simulink model "Model_B"  (R2024b)
settings: Solver=ode15s  StartTime=0.0  StopTime=3  MaxStep=0.00020000000000000001  MinStep=1e-9  RelTol=9.9999999999999995e-08  AbsTol=1.0000000000000001e-09
PostLoadFcn:
  | f=fileparts(get_param(bdroot,'FileName'));addpath(f,fullfile(f,'..','ModelA'));
InitFcn:
  | Model_B_initialize(bdroot);
model workspace (MAT data in the model file):
  ic.Vnom = 1
  ic.referenceA.x0 = [0.0487207667186; 0; 1.03532101344; 2.70319926687e-24]
  ic.referenceA.V0 = 0.998847335682-0.048i
  ic.referenceA.Vnom = 1
  ic.referenceA.network = [0.998847335682; -0.048; 1; 1; 0.414093240727; 1.04542083745; 0.30480276799; 39666.4759309; 0; 1.22124532709e-15; 12.929734979; 0]
  ic.referenceA.residual = 1.21569421196e-14
  ic.referenceA.eigenvalues = [-0.599279843882+14.9008401777i; -0.599279843882-14.9008401777i; -5.25574712927+0i; -62.8318530718+0i]
  ic.x0 = [0.200769576757; 0; 1.03524949847; 1.07980110806e-24; 0; 0; 5.29655064166e-05; -1.84134158413e-05; 0.965950721518; -0.335811993898; 1.03524949847; -1.04303465943e-24; 0.965950721518; -0.404138460797]
  ic.y0 = [0.95847228581; -0.0493156664303; 0.959740151093; 0.95847228581; -0.0493156664303; 0.959740151093; 0.969798975745; -0.142871915924; 205.357045203; 0; 5.55111512313e-17; 2.71009793582; 0.994518056541; 0.144286965879; 1.04708580923; 1.03524949847; -1.04303465943e-24; 0.965950721518; -0.335811993898; 1.09045105116; 0.143213548258; 0; 0; 0; 0; 0]
  ic.residual = 1.79625227647e-12
  ic.Jacobian = [0  376.991118431  0  0  0  0  0  0  0  0  0  0  0  0; 0  -1.19464797706  -0.19232851257  0  0  0  0  0  0  0  0  0  -0.206126453186  0; 0  0  -5.03367820511  0  0  0  0  0  0  0  0  0  0  0.0862707915375; 0  0  0  -62.8318530718  0  0  0  0  0  0  0  0  0  0; 0  0  1.00000000001  -0.404138460697  0  0  0  0  0  0  -1.00000000001  0  0  0; 0  0  0  -0.965950721518  0  0  0  0  0  0  0  -1  -1.07980110809e-24  0; 0  0  0.00483446526552  -0.00195379334933  0.00172522007791  0  0  0  -1.00000000002  0  -0.00483446526552  -0.0660000000208  1.00000000002  0; 0  0.068326466901  0  -0.00466985516923  0  0.00172522013342  0  0  0  -1.00000000001  0.0660000000111  -0.00483446527255  0  0.999999999989; 0  -4.35983562251e-08  80.8855152144  -32.6889475634  28.8646844728  0  229177.356794  0  -16743.582286  7.83314234475e-08  -80.8855152144  -1104.24705101  16731.0159154  0; 0  1143.17120514  0  -78.1314211307  0  28.8646855192  0  229177.356794  0  -16743.5822859  1104.24705059  -80.8855154117  0  16731.0159149; 0  -3.93214802855e-22  0  0  0  0  0  0  5711.98664298  0  0  376.991118431  -5711.98664298  0; 0  -390.279866255  0  0  0  0  0  0  0  5711.98664293  -376.991118436  0  0  -5711.98664283; 1330.57569228  -152.356610329  0  0  0  0  0  0  0  0  2513.27412289  0  -171.394474141  1449.18654791; 2276.91091453  -364.154842827  0  0  0  0  0  0  0  0  0  2513.27412287  -1153.65532456  146.261732879]
  ic.eigenvalues = [-15794.2331673+321.061333144i; -15794.2331673-321.061333144i; -929.230478464+1324.15474358i; -929.230478464-1324.15474358i; -1.19066242403+12.8639119334i; -1.19066242403-12.8639119334i; -18.1217144526+11.723297357i; -18.1217144526-11.723297357i; -5.2077916342+0i; -13.5205584626+0.471109259308i; -13.5205584626-0.471109259308i; -0.361420035876+0i; -0.363265507273+0i; -62.8318530718+0i]
  networkParameters = [0.1; 0; 0.24; 1.2; 0.3; 1; 0; 0.01; 0; 1; 1]
  p.baseMVA = 100
  p.freq = 60
  p.M = 5.0224
  p.D = 6
  p.K = 12
  p.Dq = 60
  p.xe = 0.1
  p.xL1 = 0
  p.xL2 = 0.24
  p.PL = 1.2
  p.QL = 0.3
  p.VS = 1
  p.thetaS = 0
  p.Pref = 1
  p.Eref = 1.03532101344
  p.Qref = 0.414093240727
  p.Ithresh = 1.1
  p.Imax = 1.5
  p.SigmaXR = 5
  p.Vmax = 1
  p.KVI = 0.283333333333
  p.omegaVI = 62.8318530718
  p.xvmax = 0.566666666667
  p.faultEnabled = 1
  p.tFault = 0.1
  p.tClear = 0.18
  p.Rf = 0.01
  p.Xf = 0
  p.faultLoadToZ = 1
  p.Vswitch = 1
  p.tStop = 3
  p.solver = 'ode15s'
  p.maxStep = 0.0002
  p.relTol = 1e-07
  p.absTol = 1e-09
  p.initTol = 1e-09
  p.residualTol = 1e-07
  p.showFigures = 1
  p.saveResults = 1
  p.outputDir = 'D:\matlab\威\威-1304-售后-200-10.20\PI优化_20261020\ModelA\Model_A_results'
  p.basekV = 345
  p.xLf = 0.15
  p.xLc = 0.15
  p.bCf = 0.066
  p.rLf = 0.005
  p.rLc = 0.005
  p.Kpv = 0.00483446524834
  p.Kiv = 0.00172522012549
  p.Kpc = 6.65705971459
  p.Kic = 91.1867729461
  p.designCurrentHz = 3000
  p.designVoltageHz = 0.5
  p.designDamping = 4
values from neighbouring files (symbols this model uses):
  ic = Model_B_initial_state(p);mw.assignin('p',p);mw.assignin('ic',ic)    [Model_B_initialize.m]
  p = mw.getVariable('p')    [Model_B_initialize.m]    (also in Model_B_parameters.m = design_Model_B_PI(p,3000,.5,4); optimize_Model_B_PI.m = p0;for j=1:4,p.(names{j})=gains(j);end; refine_PI_local.m = p0;for gainIndex=1:4,p.(names{gainIndex})=gains(gainIndex);e)
settings Model: Creator=Administrator  LastModifiedBy=Administrator
settings DataIOCC: SaveOutput=off  SignalLogging=off
settings DebuggingCC: AlgebraicLoopMsg=error  MinStepSizeMsg=error

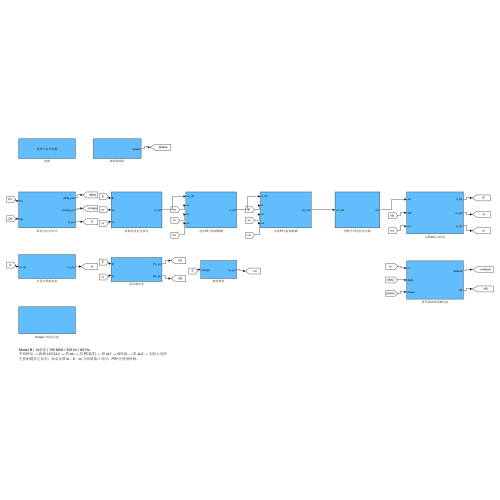
[thumbnail: Simulink's stored preview of the top-level diagram]
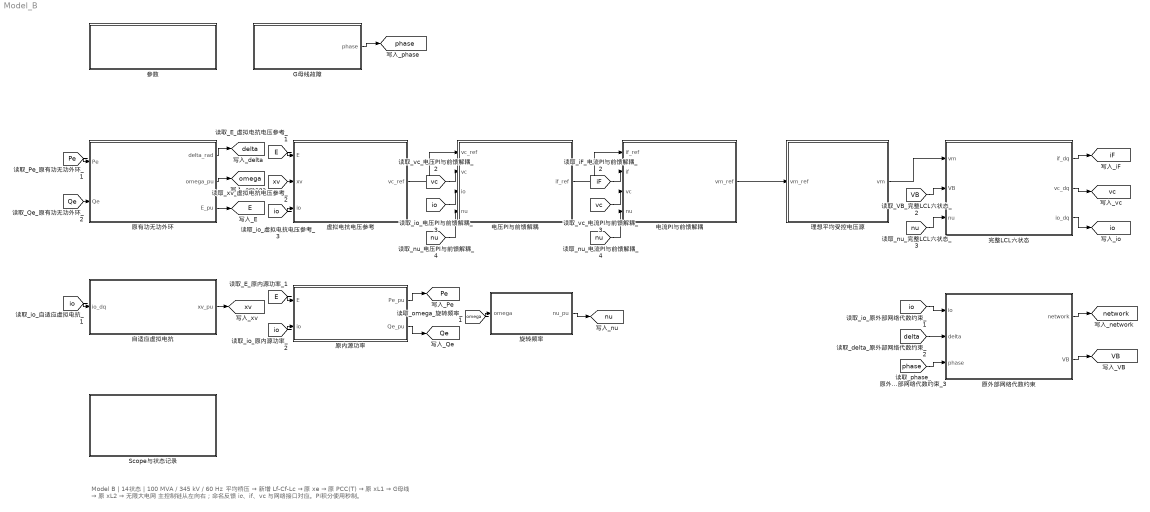
== system Model_B ==
  note: Model B | 14状态 | 100 MVA / 345 kV / 60 Hz
      | 平均桥压 → 新增 Lf-Cf-Lc → 原 xe → 原 PCC(T) → 原 xL1 → G母线 → 原 xL2 → 无限大电网
      | 主控制链从左向右；命名反馈 io、if、vc 与网络接口对应。PI积分使用秒制。
  G母线故障 : Subsystem
  Scope与状态记录 : Subsystem
  原内源功率 : Subsystem
  原外部网络代数约束 : Subsystem
  原有功无功外环 : Subsystem
  参数 : Subsystem  mask{baseMVA=100, freq=60, M=5.0224000000000002, D=6, K=12, Dq=60, xe=0.10000000000000001, xL1=0, xL2=0.23999999999999999, PL=1.2, QL=0.29999999999999999, VS=1, thetaS=0, Pref=1, Eref=1.0353210134405997, Qref=0.41409324072705855, Ithresh=1.1000000000000001, Imax=1.5, SigmaXR=5, Vmax=1, KVI=0.28333333333333344, omegaVI=62.831853071795862, xvmax=0.56666666666666676, faultEnabled=1, tFault=0.10000000000000001, tClear=0.17999999999999999, Rf=0.01, Xf=0, faultLoadToZ=1, Vswitch=1, tStop=3, maxStep=0.00020000000000000001, relTol=9.9999999999999995e-08, absTol=1.0000000000000001e-09, initTol=1.0000000000000001e-09, residualTol=9.9999999999999995e-08, basekV=345, xLf=0.14999999999999999, xLc=0.14999999999999999, bCf=0.066000000000000003, rLf=0.0050000000000000001, rLc=0.0050000000000000001, Kpv=0.0048344652483415206, Kiv=0.0017252201254877612, Kpc=6.6570597145874624, Kic=91.186772946123014}
      mask help: 标幺量与秒制。修改参数后直接运行，初值自动重新求解。
      mask Display: disp('系统与内环参数')
  完整LCL六状态 : Subsystem
  旋转频率 : Subsystem
  理想平均受控电压源 : Subsystem
  电压PI与前馈解耦 : Subsystem
  电流PI与前馈解耦 : Subsystem
  自适应虚拟电抗 : Subsystem
  虚拟电抗电压参考 : Subsystem
  tag scope: E=global, Pe=global, Qe=global, VB=global, delta=global, iF=global, io=global, network=global, nu=global, omega=global, phase=global, vc=global, xv=global
  wires:
  G母线故障/1(phase) -> [phase]
  [Pe] -> 原有功无功外环/1(Pe)
  [Qe] -> 原有功无功外环/2(Qe)
  原有功无功外环/1(delta_rad) -> [delta]
  原有功无功外环/2(omega_pu) -> [omega]
  原有功无功外环/3(E_pu) -> [E]
  [io] -> 自适应虚拟电抗/1(io_dq)
  自适应虚拟电抗/1(xv_pu) -> [xv]
  [E] -> 虚拟电抗电压参考/1(E)
  [xv] -> 虚拟电抗电压参考/2(xv)
  [io] -> 虚拟电抗电压参考/3(io)
  虚拟电抗电压参考/1(vc_ref) -> 电压PI与前馈解耦/1(vc_ref)
  [vc] -> 电压PI与前馈解耦/2(vc)
  [io] -> 电压PI与前馈解耦/3(io)
  [nu] -> 电压PI与前馈解耦/4(nu)
  电压PI与前馈解耦/1(if_ref) -> 电流PI与前馈解耦/1(if_ref)
  [iF] -> 电流PI与前馈解耦/2(if)
  [vc] -> 电流PI与前馈解耦/3(vc)
  [nu] -> 电流PI与前馈解耦/4(nu)
  电流PI与前馈解耦/1(vm_ref) -> 理想平均受控电压源/1(vm_ref)
  理想平均受控电压源/1(vm) -> 完整LCL六状态/1(vm)
  [VB] -> 完整LCL六状态/2(VB)
  [nu] -> 完整LCL六状态/3(nu)
  完整LCL六状态/1(if_dq) -> [iF]
  完整LCL六状态/2(vc_dq) -> [vc]
  完整LCL六状态/3(io_dq) -> [io]
  [io] -> 原外部网络代数约束/1(io)
  [delta] -> 原外部网络代数约束/2(delta)
  [phase] -> 原外部网络代数约束/3(phase)
  原外部网络代数约束/1(network) -> [network]
  原外部网络代数约束/2(VB) -> [VB]
  [E] -> 原内源功率/1(E)
  [io] -> 原内源功率/2(io)
  原内源功率/1(Pe_pu) -> [Pe]
  原内源功率/2(Qe_pu) -> [Qe]
  [omega] -> 旋转频率/1(omega)
  旋转频率/1(nu_pu) -> [nu]

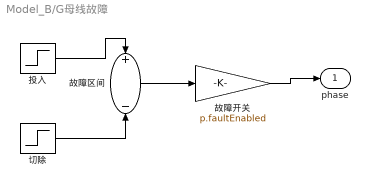
== system Model_B/G母线故障 ==
  切除 : Step  Time=p.tClear  SampleTime=0
  投入 : Step  Time=p.tFault  SampleTime=0
  故障区间 : Sum  Inputs=+-
  故障开关 : Gain  Gain=p.faultEnabled
  phase : Outport
  wires:
  投入/1 -> 故障区间/1
  切除/1 -> 故障区间/2
  故障区间/1 -> 故障开关/1
  故障开关/1 -> phase/1

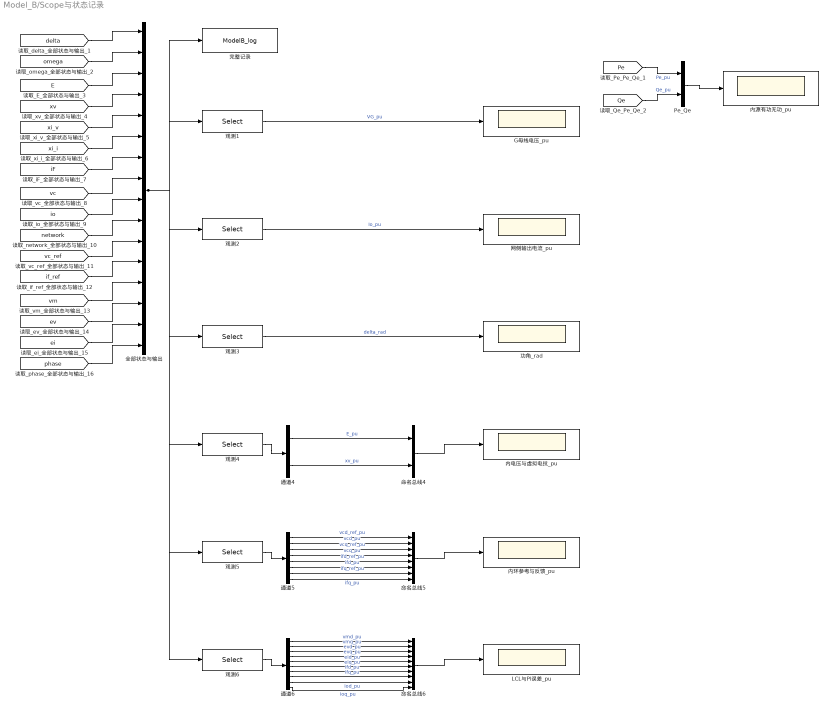
== system Model_B/Scope与状态记录 ==
  G母线电压_pu : Scope
  LCL与PI误差_pu : Scope
  Pe_Qe : BusCreator  Inputs=2
  全部状态与输出 : Mux  Inputs=16
  内源有功无功_pu : Scope
  内环参考与反馈_pu : Scope
  内电压与虚拟电抗_pu : Scope
  功角_rad : Scope
  命名总线4 : BusCreator  Inputs=2
  命名总线5 : BusCreator  Inputs=8
  命名总线6 : BusCreator  Inputs=10
  完整记录 : ToWorkspace  VariableName=ModelB_log  SaveFormat=Timeseries  SampleTime=-1
  网侧输出电流_pu : Scope
  观测1 : Selector  IndexOptions=Index vector (dialog)  Indices=17  OutputSizes=1
  观测2 : Selector  IndexOptions=Index vector (dialog)  Indices=29  OutputSizes=1
  观测3 : Selector  IndexOptions=Index vector (dialog)  Indices=1  OutputSizes=1
  观测4 : Selector  IndexOptions=Index vector (dialog)  Indices=[3 4]  OutputSizes=1
  观测5 : Selector  IndexOptions=Index vector (dialog)  Indices=[30 11 31 12 32 9 33 10]  OutputSizes=1
  观测6 : Selector  IndexOptions=Index vector (dialog)  Indices=[34 35 36 37 38 39 9 10 13 14]  OutputSizes=1
  通道4 : Demux  Outputs=2
  通道5 : Demux  Outputs=8
  通道6 : Demux  Outputs=10
  wires:
  [delta] -> 全部状态与输出/1
  [omega] -> 全部状态与输出/2
  [E] -> 全部状态与输出/3
  [xv] -> 全部状态与输出/4
  [xi_v] -> 全部状态与输出/5
  [xi_i] -> 全部状态与输出/6
  [iF] -> 全部状态与输出/7
  [vc] -> 全部状态与输出/8
  [io] -> 全部状态与输出/9
  [network] -> 全部状态与输出/10
  [vc_ref] -> 全部状态与输出/11
  [if_ref] -> 全部状态与输出/12
  [vm] -> 全部状态与输出/13
  [ev] -> 全部状态与输出/14
  [ei] -> 全部状态与输出/15
  [phase] -> 全部状态与输出/16
  全部状态与输出/1 -> 完整记录/1, 观测1/1, 观测2/1, 观测3/1, 观测4/1, 观测5/1, 观测6/1
  观测1/1 -> G母线电压_pu/1  "VG_pu"
  观测2/1 -> 网侧输出电流_pu/1  "Io_pu"
  观测3/1 -> 功角_rad/1  "delta_rad"
  观测4/1 -> 通道4/1
  通道4/1 -> 命名总线4/1  "E_pu"
  通道4/2 -> 命名总线4/2  "xv_pu"
  命名总线4/1 -> 内电压与虚拟电抗_pu/1
  观测5/1 -> 通道5/1
  通道5/1 -> 命名总线5/1  "vcd_ref_pu"
  通道5/2 -> 命名总线5/2  "vcd_pu"
  通道5/3 -> 命名总线5/3  "vcq_ref_pu"
  通道5/4 -> 命名总线5/4  "vcq_pu"
  通道5/5 -> 命名总线5/5  "ifd_ref_pu"
  通道5/6 -> 命名总线5/6  "ifd_pu"
  通道5/7 -> 命名总线5/7  "ifq_ref_pu"
  通道5/8 -> 命名总线5/8  "ifq_pu"
  命名总线5/1 -> 内环参考与反馈_pu/1
  观测6/1 -> 通道6/1
  通道6/1 -> 命名总线6/1  "vmd_pu"
  通道6/2 -> 命名总线6/2  "vmq_pu"
  通道6/3 -> 命名总线6/3  "evd_pu"
  通道6/4 -> 命名总线6/4  "evq_pu"
  通道6/5 -> 命名总线6/5  "eid_pu"
  通道6/6 -> 命名总线6/6  "eiq_pu"
  通道6/7 -> 命名总线6/7  "ifd_pu"
  通道6/8 -> 命名总线6/8  "ifq_pu"
  通道6/9 -> 命名总线6/9  "iod_pu"
  通道6/10 -> 命名总线6/10  "ioq_pu"
  命名总线6/1 -> LCL与PI误差_pu/1
  [Pe] -> Pe_Qe/1  "Pe_pu"
  [Qe] -> Pe_Qe/2  "Qe_pu"
  Pe_Qe/1 -> 内源有功无功_pu/1

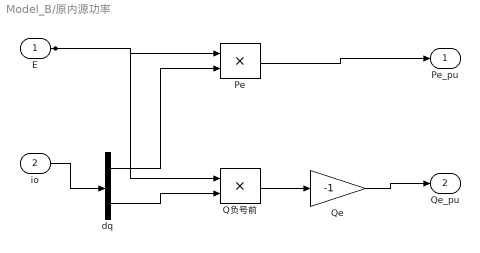
== system Model_B/原内源功率 ==
  E : Inport
  io : Inport  Port=2
  Pe : Product
  Qe : Gain  Gain=-1
  Q负号前 : Product
  dq : Demux  Outputs=2
  Pe_pu : Outport
  Qe_pu : Outport  Port=2
  wires:
  io/1 -> dq/1
  E/1 -> Pe/1, Q负号前/1
  dq/1 -> Pe/2
  dq/2 -> Q负号前/2
  Q负号前/1 -> Qe/1
  Pe/1 -> Pe_pu/1
  Qe/1 -> Qe_pu/1

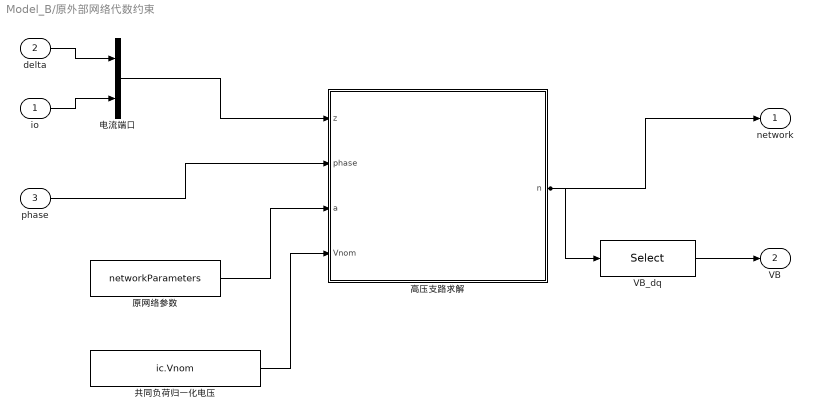
== system Model_B/原外部网络代数约束 ==
  io : Inport
  delta : Inport  Port=2
  phase : Inport  Port=3
  VB_dq : Selector  IndexOptions=Index vector (dialog)  Indices=[7 8]  OutputSizes=1
  共同负荷归一化电压 : Constant  Value=ic.Vnom
  原网络参数 : Constant  Value=networkParameters
  电流端口 : Mux  Inputs=2
  高压支路求解 : MATLAB Function  TreatAsAtomicUnit=on
  network : Outport
  VB : Outport  Port=2
  wires:
  delta/1 -> 电流端口/1
  io/1 -> 电流端口/2
  电流端口/1 -> 高压支路求解/1(z)
  phase/1 -> 高压支路求解/2(phase)
  原网络参数/1 -> 高压支路求解/3(a)
  共同负荷归一化电压/1 -> 高压支路求解/4(Vnom)
  高压支路求解/1(n) -> VB_dq/1, network/1
  VB_dq/1 -> VB/1

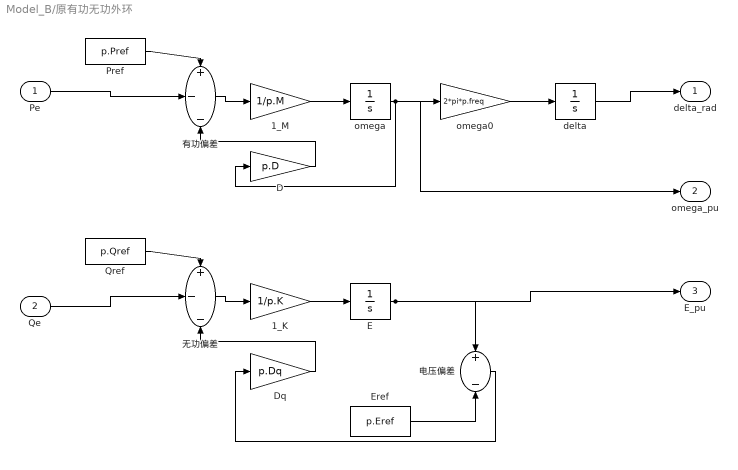
== system Model_B/原有功无功外环 ==
  Pe : Inport
  Qe : Inport  Port=2
  1_K : Gain  Gain=1/p.K
  1_M : Gain  Gain=1/p.M
  D : Gain  Gain=p.D
  Dq : Gain  Gain=p.Dq
  E : Integrator  InitialCondition=ic.x0(3)
  Eref : Constant  Value=p.Eref
  Pref : Constant  Value=p.Pref
  Qref : Constant  Value=p.Qref
  delta : Integrator  InitialCondition=ic.x0(1)
  omega : Integrator  InitialCondition=ic.x0(2)
  omega0 : Gain  Gain=2*pi*p.freq
  无功偏差 : Sum  Inputs=+--
  有功偏差 : Sum  Inputs=+--
  电压偏差 : Sum  Inputs=+-
  delta_rad : Outport
  omega_pu : Outport  Port=2
  E_pu : Outport  Port=3
  wires:
  Pref/1 -> 有功偏差/1
  Pe/1 -> 有功偏差/2
  D/1 -> 有功偏差/3
  有功偏差/1 -> 1_M/1
  1_M/1 -> omega/1
  omega/1 -> D/1, omega0/1, omega_pu/1
  omega0/1 -> delta/1
  Qref/1 -> 无功偏差/1
  Qe/1 -> 无功偏差/2
  Dq/1 -> 无功偏差/3
  无功偏差/1 -> 1_K/1
  1_K/1 -> E/1
  E/1 -> 电压偏差/1, E_pu/1
  Eref/1 -> 电压偏差/2
  电压偏差/1 -> Dq/1
  delta/1 -> delta_rad/1

== system Model_B/参数 ==

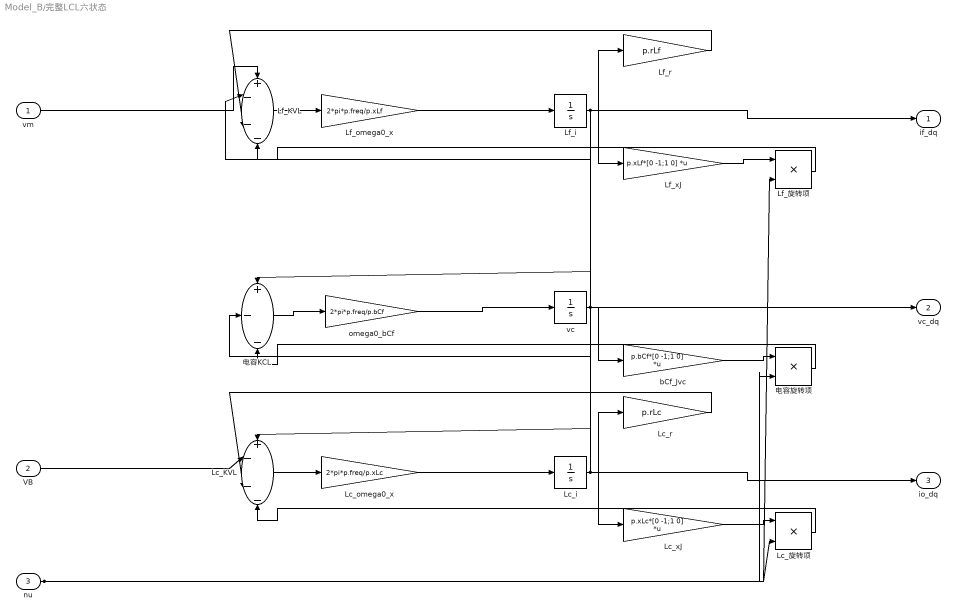
== system Model_B/完整LCL六状态 ==
  vm : Inport
  VB : Inport  Port=2
  nu : Inport  Port=3
  Lc_KVL : Sum  Inputs=+---
  Lc_i : Integrator  InitialCondition=ic.x0(13:14)
  Lc_omega0_x : Gain  Gain=2*pi*p.freq/p.xLc
  Lc_r : Gain  Gain=p.rLc
  Lc_xJ : Gain  Gain=p.xLc*[0 -1;1 0]  Multiplication=Matrix(K*u)
  Lc_旋转项 : Product
  Lf_KVL : Sum  Inputs=+---
  Lf_i : Integrator  InitialCondition=ic.x0(9:10)
  Lf_omega0_x : Gain  Gain=2*pi*p.freq/p.xLf
  Lf_r : Gain  Gain=p.rLf
  Lf_xJ : Gain  Gain=p.xLf*[0 -1;1 0]  Multiplication=Matrix(K*u)
  Lf_旋转项 : Product
  bCf_Jvc : Gain  Gain=p.bCf*[0 -1;1 0]  Multiplication=Matrix(K*u)
  omega0_bCf : Gain  Gain=2*pi*p.freq/p.bCf
  vc : Integrator  InitialCondition=ic.x0(11:12)
  电容KCL : Sum  Inputs=+--
  电容旋转项 : Product
  if_dq : Outport
  vc_dq : Outport  Port=2
  io_dq : Outport  Port=3
  wires:
  Lf_KVL/1 -> Lf_omega0_x/1
  Lf_omega0_x/1 -> Lf_i/1
  Lf_i/1 -> Lf_r/1, Lf_xJ/1, 电容KCL/1, if_dq/1
  Lf_r/1 -> Lf_KVL/3
  Lf_xJ/1 -> Lf_旋转项/1
  nu/1 -> Lf_旋转项/2, Lc_旋转项/2, 电容旋转项/2
  Lf_旋转项/1 -> Lf_KVL/4
  Lc_KVL/1 -> Lc_omega0_x/1
  Lc_omega0_x/1 -> Lc_i/1
  Lc_i/1 -> Lc_r/1, Lc_xJ/1, 电容KCL/2, io_dq/1
  Lc_r/1 -> Lc_KVL/3
  Lc_xJ/1 -> Lc_旋转项/1
  Lc_旋转项/1 -> Lc_KVL/4
  电容KCL/1 -> omega0_bCf/1
  omega0_bCf/1 -> vc/1
  vc/1 -> bCf_Jvc/1, Lf_KVL/2, Lc_KVL/1, vc_dq/1
  bCf_Jvc/1 -> 电容旋转项/1
  vm/1 -> Lf_KVL/1
  VB/1 -> Lc_KVL/2
  电容旋转项/1 -> 电容KCL/3

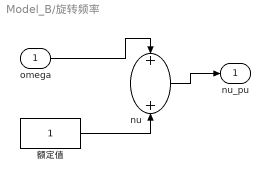
== system Model_B/旋转频率 ==
  omega : Inport
  nu : Sum
  额定值 : Constant
  nu_pu : Outport
  wires:
  omega/1 -> nu/1
  额定值/1 -> nu/2
  nu/1 -> nu_pu/1

== system Model_B/理想平均受控电压源 ==
  vm_ref : Inport
  vm等于vm_ref : Gain
  vm : Outport
  tag scope: vm=global
  wires:
  vm_ref/1 -> vm等于vm_ref/1
  vm等于vm_ref/1 -> vm/1, [vm]

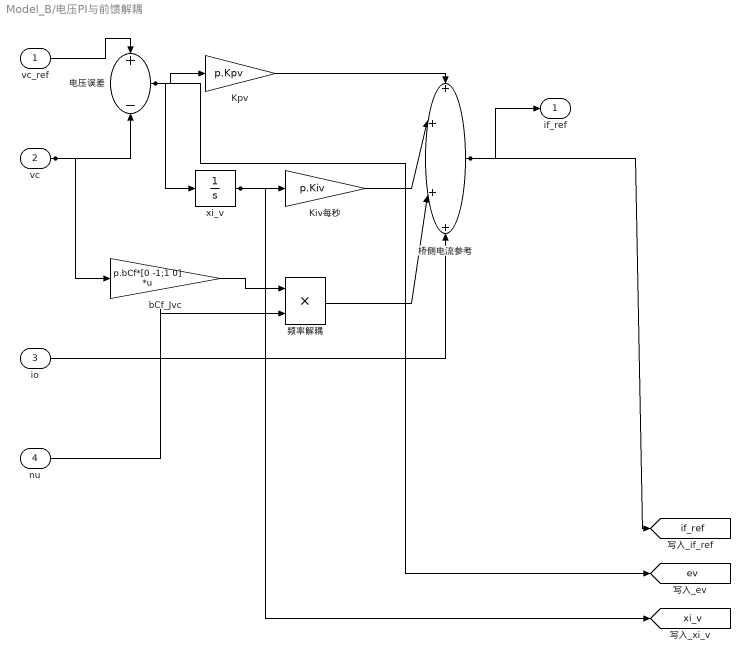
== system Model_B/电压PI与前馈解耦 ==
  vc_ref : Inport
  vc : Inport  Port=2
  io : Inport  Port=3
  nu : Inport  Port=4
  Kiv每秒 : Gain  Gain=p.Kiv
  Kpv : Gain  Gain=p.Kpv
  bCf_Jvc : Gain  Gain=p.bCf*[0 -1;1 0]  Multiplication=Matrix(K*u)
  xi_v : Integrator  InitialCondition=ic.x0(5:6)
  桥侧电流参考 : Sum  Inputs=++++
  电压误差 : Sum  Inputs=+-
  频率解耦 : Product
  if_ref : Outport
  tag scope: ev=global, if_ref=global, xi_v=global
  wires:
  vc_ref/1 -> 电压误差/1
  vc/1 -> 电压误差/2, bCf_Jvc/1
  电压误差/1 -> Kpv/1, xi_v/1, [ev]
  xi_v/1 -> Kiv每秒/1, [xi_v]
  bCf_Jvc/1 -> 频率解耦/1
  nu/1 -> 频率解耦/2
  Kpv/1 -> 桥侧电流参考/1
  Kiv每秒/1 -> 桥侧电流参考/2
  频率解耦/1 -> 桥侧电流参考/3
  io/1 -> 桥侧电流参考/4
  桥侧电流参考/1 -> if_ref/1, [if_ref]

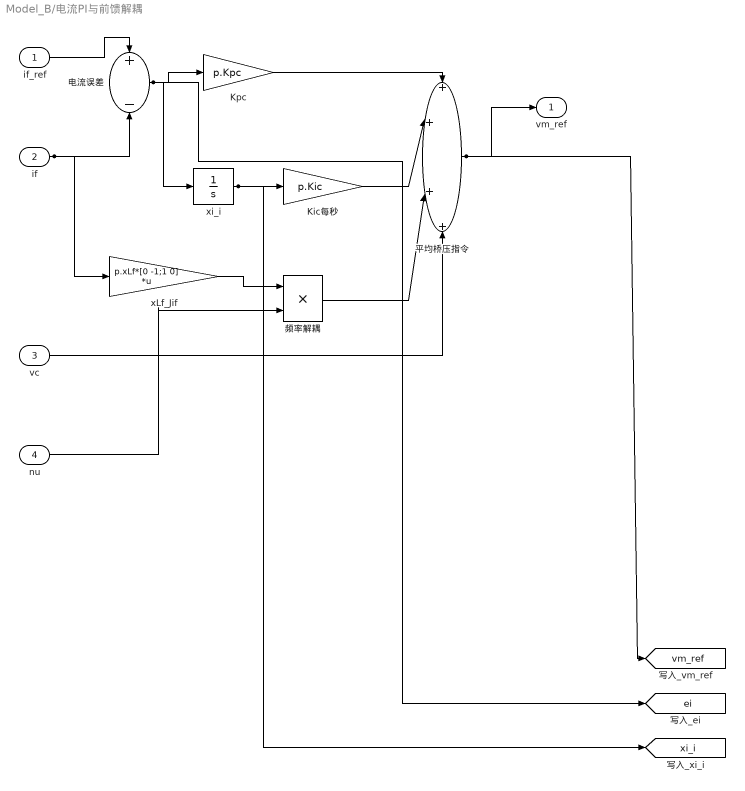
== system Model_B/电流PI与前馈解耦 ==
  if_ref : Inport
  if : Inport  Port=2
  vc : Inport  Port=3
  nu : Inport  Port=4
  Kic每秒 : Gain  Gain=p.Kic
  Kpc : Gain  Gain=p.Kpc
  xLf_Jif : Gain  Gain=p.xLf*[0 -1;1 0]  Multiplication=Matrix(K*u)
  xi_i : Integrator  InitialCondition=ic.x0(7:8)
  平均桥压指令 : Sum  Inputs=++++
  电流误差 : Sum  Inputs=+-
  频率解耦 : Product
  vm_ref : Outport
  tag scope: ei=global, vm_ref=global, xi_i=global
  wires:
  if_ref/1 -> 电流误差/1
  if/1 -> 电流误差/2, xLf_Jif/1
  电流误差/1 -> Kpc/1, xi_i/1, [ei]
  xi_i/1 -> Kic每秒/1, [xi_i]
  xLf_Jif/1 -> 频率解耦/1
  nu/1 -> 频率解耦/2
  Kpc/1 -> 平均桥压指令/1
  Kic每秒/1 -> 平均桥压指令/2
  频率解耦/1 -> 平均桥压指令/3
  vc/1 -> 平均桥压指令/4
  平均桥压指令/1 -> vm_ref/1, [vm_ref]

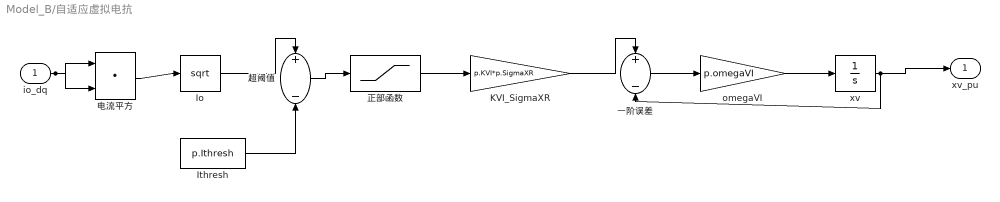
== system Model_B/自适应虚拟电抗 ==
  io_dq : Inport
  Io : Sqrt
  Ithresh : Constant  Value=p.Ithresh
  KVI_SigmaXR : Gain  Gain=p.KVI*p.SigmaXR
  omegaVI : Gain  Gain=p.omegaVI
  xv : Integrator  InitialCondition=ic.x0(4)
  一阶误差 : Sum  Inputs=+-
  正部函数 : Saturate  UpperLimit=inf  LowerLimit=0
  电流平方 : DotProduct  OutDataTypeStr=Inherit: Inherit via internal rule
  超阈值 : Sum  Inputs=+-
  xv_pu : Outport
  wires:
  io_dq/1 -> 电流平方/1, 电流平方/2
  电流平方/1 -> Io/1
  Io/1 -> 超阈值/1
  Ithresh/1 -> 超阈值/2
  超阈值/1 -> 正部函数/1
  正部函数/1 -> KVI_SigmaXR/1
  KVI_SigmaXR/1 -> 一阶误差/1
  一阶误差/1 -> omegaVI/1
  omegaVI/1 -> xv/1
  xv/1 -> 一阶误差/2, xv_pu/1

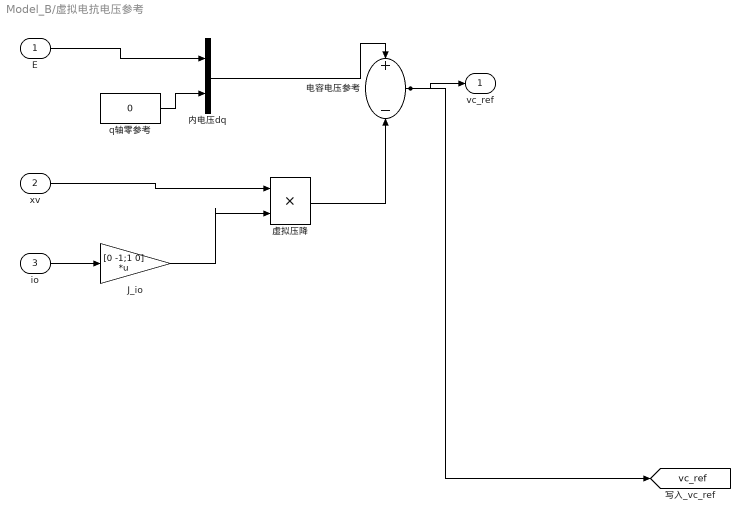
== system Model_B/虚拟电抗电压参考 ==
  E : Inport
  xv : Inport  Port=2
  io : Inport  Port=3
  J_io : Gain  Gain=[0 -1;1 0]  Multiplication=Matrix(K*u)
  q轴零参考 : Constant  Value=0
  内电压dq : Mux  Inputs=2
  电容电压参考 : Sum  Inputs=+-
  虚拟压降 : Product
  vc_ref : Outport
  tag scope: vc_ref=global
  wires:
  E/1 -> 内电压dq/1
  q轴零参考/1 -> 内电压dq/2
  io/1 -> J_io/1
  J_io/1 -> 虚拟压降/2
  xv/1 -> 虚拟压降/1
  内电压dq/1 -> 电容电压参考/1
  虚拟压降/1 -> 电容电压参考/2
  电容电压参考/1 -> vc_ref/1, [vc_ref]

== matlab function Model_B/原外部网络代数约束/高压支路求解 ==
  data: z input; n output; phase input; a input; Vnom input
function n=Model_B_network(z,phase,a,Vnom)
%#codegen
% z=[delta;iod;ioq]；电流端口连接原外部准稳态网络。
Io=complex(z(2),z(3))*exp(1i*z(1));Vs=a(6)*exp(1i*a(7));
Y=1/(1i*a(3));if phase==1,Y=Y+1/complex(a(8),a(9));end
A=Io+Vs/(1i*a(3));S=complex(a(4),a(5));
aa=abs(Y)^2;b=abs(A)^2-2*real(Y*S);disc=b*b-4*aa*abs(S)^2;
exists=disc>0 && b>0 && abs(A)>0;Vcp=complex(0,0);
if exists,u=(b+sqrt(disc))/(2*aa);Vcp=conj((Y*u+conj(S))/A);end
V=Vcp;loadZ=false;
if phase==1 && a(10)~=0
    Vz=A/(Y+conj(S)/(Vnom*Vnom));
    if (~exists || abs(Vcp)<a(11)) && abs(Vz)<a(11),V=Vz;loadZ=true;end
end
assert(~(disc==0 && b>0 && abs(A)>0 && ~loadZ),'Model_B_DAE_SINGULAR: algebraic branches meet.');
assert(exists || loadZ,'Model_B_DAE_NO_REAL_SOLUTION: original external network has no regular high-voltage solution.');
assert(abs(V)>0,'Model_B_DAE_ZERO_VOLTAGE');
Seff=S;if loadZ,Seff=S*abs(V)^2/(Vnom*Vnom);end
g=V*conj(A-Y*V)-Seff;
vr=real(V);vi=imag(V);G=real(Y);B=imag(Y);
J=[real(A)-2*G*vr,imag(A)-2*G*vi;-imag(A)+2*B*vr,real(A)+2*B*vi];
if loadZ,J=J-2/(Vnom*Vnom)*[a(4)*vr,a(4)*vi;a(5)*vr,a(5)*vi];end
sv=svd(J);
VT=V+1i*a(2)*Io;VB=(VT+1i*a(1)*Io)*exp(-1i*z(1));Spcc=VT*conj(Io);
n=[real(V);imag(V);abs(V);real(VT);imag(VT);abs(VT);real(VB);imag(VB); ...
    disc;double(loadZ);max(abs([real(g);imag(g)]));min(sv);real(Spcc);imag(Spcc);abs(Io)];
end
